simulink model "induction_motor_foc"  (R2021a)
settings: Solver=FixedStepAuto  StartTime=0.0  StopTime=3  FixedStep=0.000001  RelTol=1e-3
values from neighbouring files (symbols this model uses):
  A1 = [-1/(ts*sig) 0 lm/(ls*tr*sig) 0;0 -1/(ts*sig) 0 lm/(ls*tr*sig);lm/(lr*ts*sig) 0 -1/(tr*sig) 0; 0 lm/(lr*ts*sig) 0 -1/(tr*sig)]    [induction_motor_parameters.m]
  A2 = [0 1 0 0; -1 0 0 0;0 0 0 1;0 0 -1 0]    [induction_motor_parameters.m]
  A3 = [0 1/sig 0 lm/(ls*sig);-1/sig 0 -lm/(ls*sig) 0;0 -lm/(lr*sig) 0 -lm*lm/(ls*lr*sig); lm/(lr*sig) 0 lm*lm/(ls*lr*sig) 0]    [induction_motor_parameters.m]
  B = [1/(ls*sig) 0 0 0;0 1/(ls*sig) 0 0; -lm/(ls*lr*sig) 0 0 0;0 -lm/(ls*lr*sig) 0 0 ]    [induction_motor_parameters.m]
  fr = 0.0015    [induction_motor_parameters.m]
  j = 0.0056    [induction_motor_parameters.m]
  KiF = 2*(Rouf^2)*lr/(lm*rr)    (= 6305.05825519)    [induction_motor_parameters.m]
  KiI = 2*(Rou^2)*ls*sig    (= 315.492957746)    [induction_motor_parameters.m]
  KiV = 2*(RouV^2)*j/p    (= 0.005054)    [induction_motor_parameters.m]
  KpF = (2*Rouf-Pr)*lr/(lm*rr)    (= 111.608411481)    [induction_motor_parameters.m]
  KpI = (2*Rou-Ps)*sig*ls    (= 1.14246478873)    [induction_motor_parameters.m]
  KpV = 12*KpV    (= 0.05484)    [induction_motor_parameters.m]
  L = [ls 0 lm 0;0 ls 0 lm;lm 0 lr 0;0 lm 0 lr]    [induction_motor_parameters.m]
  lm = 0.069    [induction_motor_parameters.m]
  lr = 0.071    [induction_motor_parameters.m]
  p = 2    [induction_motor_parameters.m]
  T = [2/3 -1/3 -1/3 ; -1/3 2/3 -1/3;-1/3 -1/3 2/3]    [induction_motor_parameters.m]
  T_dent = t/m    (= 0.000952380952381)    [induction_motor_parameters.m]
  tr = lr/rr    (= 0.0870098039216)    [induction_motor_parameters.m]
libraries: simulink x4, pid_lib x4, spsdq0toabcLib x2, spsabctodq0Lib x1

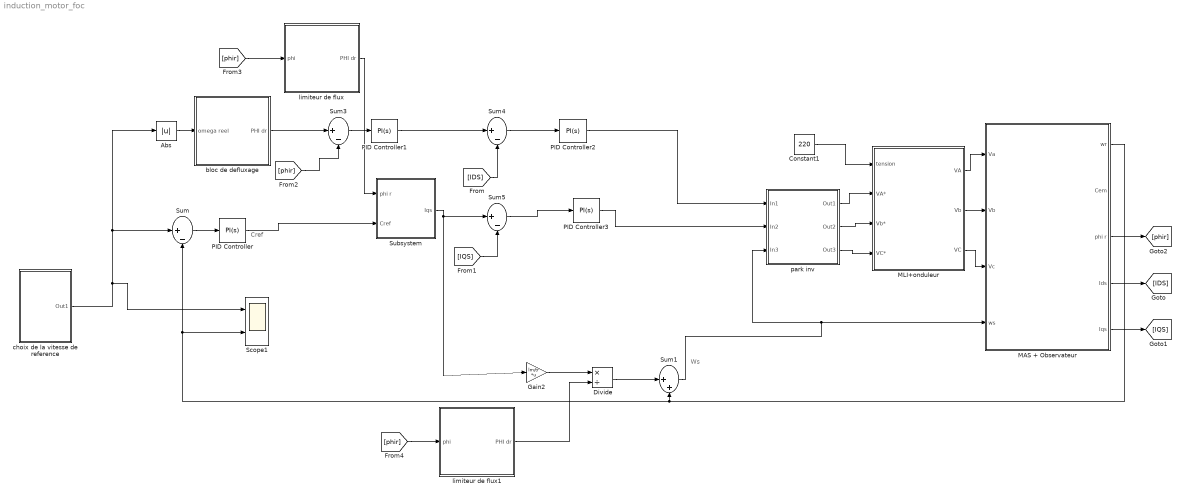
== system induction_motor_foc ==
  note: Ws
  note: Cref
  Abs : Abs
  Constant1 : Constant  Value=220
  Divide : Product  Inputs=*/
  Gain2 : Gain  Gain=lm/tr  Multiplication=Matrix(K*u)
  MAS + Observateur : Subsystem
  MLI+onduleur : Subsystem
  PID Controller : pid_lib/PID Controller  Controller=PI  Form=Parallel  TimeDomain=Continuous-time  UseExternalTs=off  SampleTime=-1  IntegratorMethod=Forward Euler  FilterMethod=Forward Euler  ControllerParametersSource=internal  P=1.7*KpV  I=KiV  D=5  UseFilter=on  N=100  TunerSelectOption=Transfer Function Based (PID Tuner App)  InitialConditionSource=internal  InitialConditionForIntegrator=0  InitialConditionForFilter=0  DifferentiatorICPrevScaledInput=0  ExternalReset=none  TrackingMode=off  Kt=1  LimitOutput=off  SatLimitsSource=internal  UpperSaturationLimit=inf  LowerSaturationLimit=-inf  LinearizeAsGain=on  AntiWindupMode=none  Kb=1  POutMin=[]  POutMax=[]  IOutMin=[]  IOutMax=[]  DOutMin=[]  DOutMax=[]  NOutMin=[]  NOutMax=[]  SumOutMin=[]  SumOutMax=[]  SaturationOutMin=[]  SaturationOutMax=[]  PParamMin=[]  PParamMax=[]  IParamMin=[]  IParamMax=[]  DParamMin=[]  DParamMax=[]  NParamMin=[]  NParamMax=[]  KbParamMin=[]  KbParamMax=[]  KtParamMin=[]  KtParamMax=[]  KbOutMin=[]  KbOutMax=[]  KtOutMin=[]  KtOutMax=[]  IntegratorOutMin=[]  IntegratorOutMax=[]  FilterOutMin=[]  FilterOutMax=[]  SumI1OutMin=[]  SumI1OutMax=[]  SumI2OutMin=[]  SumI2OutMax=[]  SumI3OutMin=[]  SumI3OutMax=[]  SumI4OutMin=[]  SumI4OutMax=[]  SumDOutMin=[]  SumDOutMax=[]  DifferentiatorOutMin=[]  DifferentiatorOutMax=[]  FilterDiffOutCoefMin=[]  FilterDiffOutCoefMax=[]  ReciprocalOutMin=[]  ReciprocalOutMax=[]  SumDenOutMin=[]  SumDenOutMax=[]  SumNumOutMin=[]  SumNumOutMax=[]  DivideOutMin=[]  DivideOutMax=[]  UdiffTsProdOutMin=[]  UdiffTsProdOutMax=[]  NTsProdOutMin=[]  NTsProdOutMax=[]  UintegralTsProdOutMin=[]  UintegralTsProdOutMax=[]  UngainTsProdOutMin=[]  UngainTsProdOutMax=[]  IntegratorContinuousStateAttributes=''  IntegratorStateMustResolveToSignalObject=off  IntegratorRTWStateStorageClass=Auto  FilterContinuousStateAttributes=''  FilterStateMustResolveToSignalObject=off  FilterRTWStateStorageClass=Auto  ParallelPVariant=InternalParameters  IdealPVariant=Disabled  IVariant=InternalParameters  DVariant=Disabled  IntegratorVariant=Continuous  SatVariant=Disabled  AWVariant=Passthrough  PCopyVariant=Disabled  TRVariant=Disabled  FdbkBlocksVariant=Forward  IdealPFdbkVariant=Disabled  SatFdbkVariant=Disabled  DerivativeFilterVariant=Disabled  NVariant=Disabled  NCopyVariant=Disabled_SignalSpec  FilterICVariant=Disabled  IntegratorICVariant=InternalICs  ExternalResetVariant=Disabled  TRSumVariant=Passthrough  SumFdbkVariant=Disabled  SumVariant=Sum_PI  TsampFilterVariant=InternalTs  TsampNgainVariant=Passthrough  TsampIntegralVariant=Passthrough  ExternalSaturationOutDataTypeStr=Inherit: Same as second input
  PID Controller1 : pid_lib/PID Controller  Controller=PI  Form=Parallel  TimeDomain=Continuous-time  UseExternalTs=off  SampleTime=-1  IntegratorMethod=Forward Euler  FilterMethod=Forward Euler  ControllerParametersSource=internal  P=KpF  I=KiF  D=0.05  UseFilter=on  N=100  TunerSelectOption=Transfer Function Based (PID Tuner App)  InitialConditionSource=internal  InitialConditionForIntegrator=0  InitialConditionForFilter=0  DifferentiatorICPrevScaledInput=0  ExternalReset=none  TrackingMode=off  Kt=1  LimitOutput=off  SatLimitsSource=internal  UpperSaturationLimit=inf  LowerSaturationLimit=-inf  LinearizeAsGain=on  AntiWindupMode=none  Kb=1  POutMin=[]  POutMax=[]  IOutMin=[]  IOutMax=[]  DOutMin=[]  DOutMax=[]  NOutMin=[]  NOutMax=[]  SumOutMin=[]  SumOutMax=[]  SaturationOutMin=[]  SaturationOutMax=[]  PParamMin=[]  PParamMax=[]  IParamMin=[]  IParamMax=[]  DParamMin=[]  DParamMax=[]  NParamMin=[]  NParamMax=[]  KbParamMin=[]  KbParamMax=[]  KtParamMin=[]  KtParamMax=[]  KbOutMin=[]  KbOutMax=[]  KtOutMin=[]  KtOutMax=[]  IntegratorOutMin=[]  IntegratorOutMax=[]  FilterOutMin=[]  FilterOutMax=[]  SumI1OutMin=[]  SumI1OutMax=[]  SumI2OutMin=[]  SumI2OutMax=[]  SumI3OutMin=[]  SumI3OutMax=[]  SumI4OutMin=[]  SumI4OutMax=[]  SumDOutMin=[]  SumDOutMax=[]  DifferentiatorOutMin=[]  DifferentiatorOutMax=[]  FilterDiffOutCoefMin=[]  FilterDiffOutCoefMax=[]  ReciprocalOutMin=[]  ReciprocalOutMax=[]  SumDenOutMin=[]  SumDenOutMax=[]  SumNumOutMin=[]  SumNumOutMax=[]  DivideOutMin=[]  DivideOutMax=[]  UdiffTsProdOutMin=[]  UdiffTsProdOutMax=[]  NTsProdOutMin=[]  NTsProdOutMax=[]  UintegralTsProdOutMin=[]  UintegralTsProdOutMax=[]  UngainTsProdOutMin=[]  UngainTsProdOutMax=[]  IntegratorContinuousStateAttributes=''  IntegratorStateMustResolveToSignalObject=off  IntegratorRTWStateStorageClass=Auto  FilterContinuousStateAttributes=''  FilterStateMustResolveToSignalObject=off  FilterRTWStateStorageClass=Auto  ParallelPVariant=InternalParameters  IdealPVariant=Disabled  IVariant=InternalParameters  DVariant=Disabled  IntegratorVariant=Continuous  SatVariant=Disabled  AWVariant=Passthrough  PCopyVariant=Disabled  TRVariant=Disabled  FdbkBlocksVariant=Forward  IdealPFdbkVariant=Disabled  SatFdbkVariant=Disabled  DerivativeFilterVariant=Disabled  NVariant=Disabled  NCopyVariant=Disabled_SignalSpec  FilterICVariant=Disabled  IntegratorICVariant=InternalICs  ExternalResetVariant=Disabled  TRSumVariant=Passthrough  SumFdbkVariant=Disabled  SumVariant=Sum_PI  TsampFilterVariant=InternalTs  TsampNgainVariant=Passthrough  TsampIntegralVariant=Passthrough  ExternalSaturationOutDataTypeStr=Inherit: Same as second input
  PID Controller2 : pid_lib/PID Controller  Controller=PI  Form=Parallel  TimeDomain=Continuous-time  UseExternalTs=off  SampleTime=-1  IntegratorMethod=Forward Euler  FilterMethod=Forward Euler  ControllerParametersSource=internal  P=KpI  I=KiI  D=0.05  UseFilter=on  N=100  TunerSelectOption=Transfer Function Based (PID Tuner App)  InitialConditionSource=internal  InitialConditionForIntegrator=0  InitialConditionForFilter=0  DifferentiatorICPrevScaledInput=0  ExternalReset=none  TrackingMode=off  Kt=1  LimitOutput=off  SatLimitsSource=internal  UpperSaturationLimit=inf  LowerSaturationLimit=-inf  LinearizeAsGain=on  AntiWindupMode=none  Kb=1  POutMin=[]  POutMax=[]  IOutMin=[]  IOutMax=[]  DOutMin=[]  DOutMax=[]  NOutMin=[]  NOutMax=[]  SumOutMin=[]  SumOutMax=[]  SaturationOutMin=[]  SaturationOutMax=[]  PParamMin=[]  PParamMax=[]  IParamMin=[]  IParamMax=[]  DParamMin=[]  DParamMax=[]  NParamMin=[]  NParamMax=[]  KbParamMin=[]  KbParamMax=[]  KtParamMin=[]  KtParamMax=[]  KbOutMin=[]  KbOutMax=[]  KtOutMin=[]  KtOutMax=[]  IntegratorOutMin=[]  IntegratorOutMax=[]  FilterOutMin=[]  FilterOutMax=[]  SumI1OutMin=[]  SumI1OutMax=[]  SumI2OutMin=[]  SumI2OutMax=[]  SumI3OutMin=[]  SumI3OutMax=[]  SumI4OutMin=[]  SumI4OutMax=[]  SumDOutMin=[]  SumDOutMax=[]  DifferentiatorOutMin=[]  DifferentiatorOutMax=[]  FilterDiffOutCoefMin=[]  FilterDiffOutCoefMax=[]  ReciprocalOutMin=[]  ReciprocalOutMax=[]  SumDenOutMin=[]  SumDenOutMax=[]  SumNumOutMin=[]  SumNumOutMax=[]  DivideOutMin=[]  DivideOutMax=[]  UdiffTsProdOutMin=[]  UdiffTsProdOutMax=[]  NTsProdOutMin=[]  NTsProdOutMax=[]  UintegralTsProdOutMin=[]  UintegralTsProdOutMax=[]  UngainTsProdOutMin=[]  UngainTsProdOutMax=[]  IntegratorContinuousStateAttributes=''  IntegratorStateMustResolveToSignalObject=off  IntegratorRTWStateStorageClass=Auto  FilterContinuousStateAttributes=''  FilterStateMustResolveToSignalObject=off  FilterRTWStateStorageClass=Auto  ParallelPVariant=InternalParameters  IdealPVariant=Disabled  IVariant=InternalParameters  DVariant=Disabled  IntegratorVariant=Continuous  SatVariant=Disabled  AWVariant=Passthrough  PCopyVariant=Disabled  TRVariant=Disabled  FdbkBlocksVariant=Forward  IdealPFdbkVariant=Disabled  SatFdbkVariant=Disabled  DerivativeFilterVariant=Disabled  NVariant=Disabled  NCopyVariant=Disabled_SignalSpec  FilterICVariant=Disabled  IntegratorICVariant=InternalICs  ExternalResetVariant=Disabled  TRSumVariant=Passthrough  SumFdbkVariant=Disabled  SumVariant=Sum_PI  TsampFilterVariant=InternalTs  TsampNgainVariant=Passthrough  TsampIntegralVariant=Passthrough  ExternalSaturationOutDataTypeStr=Inherit: Same as second input
  PID Controller3 : pid_lib/PID Controller  Controller=PI  Form=Parallel  TimeDomain=Continuous-time  UseExternalTs=off  SampleTime=-1  IntegratorMethod=Forward Euler  FilterMethod=Forward Euler  ControllerParametersSource=internal  P=KpI  I=KiI  D=0.05  UseFilter=on  N=100  TunerSelectOption=Transfer Function Based (PID Tuner App)  InitialConditionSource=internal  InitialConditionForIntegrator=0  InitialConditionForFilter=0  DifferentiatorICPrevScaledInput=0  ExternalReset=none  TrackingMode=off  Kt=1  LimitOutput=off  SatLimitsSource=internal  UpperSaturationLimit=inf  LowerSaturationLimit=-inf  LinearizeAsGain=on  AntiWindupMode=none  Kb=1  POutMin=[]  POutMax=[]  IOutMin=[]  IOutMax=[]  DOutMin=[]  DOutMax=[]  NOutMin=[]  NOutMax=[]  SumOutMin=[]  SumOutMax=[]  SaturationOutMin=[]  SaturationOutMax=[]  PParamMin=[]  PParamMax=[]  IParamMin=[]  IParamMax=[]  DParamMin=[]  DParamMax=[]  NParamMin=[]  NParamMax=[]  KbParamMin=[]  KbParamMax=[]  KtParamMin=[]  KtParamMax=[]  KbOutMin=[]  KbOutMax=[]  KtOutMin=[]  KtOutMax=[]  IntegratorOutMin=[]  IntegratorOutMax=[]  FilterOutMin=[]  FilterOutMax=[]  SumI1OutMin=[]  SumI1OutMax=[]  SumI2OutMin=[]  SumI2OutMax=[]  SumI3OutMin=[]  SumI3OutMax=[]  SumI4OutMin=[]  SumI4OutMax=[]  SumDOutMin=[]  SumDOutMax=[]  DifferentiatorOutMin=[]  DifferentiatorOutMax=[]  FilterDiffOutCoefMin=[]  FilterDiffOutCoefMax=[]  ReciprocalOutMin=[]  ReciprocalOutMax=[]  SumDenOutMin=[]  SumDenOutMax=[]  SumNumOutMin=[]  SumNumOutMax=[]  DivideOutMin=[]  DivideOutMax=[]  UdiffTsProdOutMin=[]  UdiffTsProdOutMax=[]  NTsProdOutMin=[]  NTsProdOutMax=[]  UintegralTsProdOutMin=[]  UintegralTsProdOutMax=[]  UngainTsProdOutMin=[]  UngainTsProdOutMax=[]  IntegratorContinuousStateAttributes=''  IntegratorStateMustResolveToSignalObject=off  IntegratorRTWStateStorageClass=Auto  FilterContinuousStateAttributes=''  FilterStateMustResolveToSignalObject=off  FilterRTWStateStorageClass=Auto  ParallelPVariant=InternalParameters  IdealPVariant=Disabled  IVariant=InternalParameters  DVariant=Disabled  IntegratorVariant=Continuous  SatVariant=Disabled  AWVariant=Passthrough  PCopyVariant=Disabled  TRVariant=Disabled  FdbkBlocksVariant=Forward  IdealPFdbkVariant=Disabled  SatFdbkVariant=Disabled  DerivativeFilterVariant=Disabled  NVariant=Disabled  NCopyVariant=Disabled_SignalSpec  FilterICVariant=Disabled  IntegratorICVariant=InternalICs  ExternalResetVariant=Disabled  TRSumVariant=Passthrough  SumFdbkVariant=Disabled  SumVariant=Sum_PI  TsampFilterVariant=InternalTs  TsampNgainVariant=Passthrough  TsampIntegralVariant=Passthrough  ExternalSaturationOutDataTypeStr=Inherit: Same as second input
  Scope1 : Scope  NumInputPorts=2
  Subsystem : Subsystem
  Sum{,3..5} (4 alike) : Sum  Inputs=|+-
  Sum1 : Sum  Inputs=|++
  bloc de defluxage : Subsystem
  choix de la vitesse de reference : Subsystem
  limiteur de flux : Subsystem
  limiteur de flux1 : Subsystem
  park inv : Subsystem
  wires:
  MLI+onduleur/1(VA) -> MAS + Observateur/1(Va)
  Sum/1 -> PID Controller/1
  [IDS] -> Sum4/2
  MAS + Observateur/5(Iqs) -> [IQS]
  Sum4/1 -> PID Controller2/1
  Divide/1 -> Sum1/1
  MLI+onduleur/3(VC) -> MAS + Observateur/3(Vc)
  Sum1/1 -> park inv/3(In3), MAS + Observateur/4(ws)
  Sum5/1 -> PID Controller3/1
  MAS + Observateur/4(Ids) -> [IDS]
  MLI+onduleur/2(Vb) -> MAS + Observateur/2(Vb)
  PID Controller3/1 -> park inv/2(In2)
  park inv/3(Out3) -> MLI+onduleur/4(VC*)
  PID Controller2/1 -> park inv/1(In1)
  Constant1/1 -> MLI+onduleur/1(tension)
  Subsystem/1(Iqs) -> Sum5/1, Gain2/1
  park inv/1(Out1) -> MLI+onduleur/2(VA*)
  bloc de defluxage/1(PHI dr) -> Sum3/1
  park inv/2(Out2) -> MLI+onduleur/3(Vb*)
  Gain2/1 -> Divide/1
  PID Controller/1 -> Subsystem/2(Cref)
  MAS + Observateur/1(wr) -> Sum1/2, Sum/2, Scope1/2
  [IQS] -> Sum5/2
  PID Controller1/1 -> Sum4/1
  Sum3/1 -> PID Controller1/1
  MAS + Observateur/3(phi r) -> [phir]
  [phir] -> Sum3/2
  [phir] -> limiteur de flux/1(phi)
  limiteur de flux/1(PHI dr) -> Subsystem/1(phi r)
  Abs/1 -> bloc de defluxage/1(omega reel)
  limiteur de flux1/1(PHI dr) -> Divide/2
  [phir] -> limiteur de flux1/1(phi)
  choix de la vitesse de reference/1(Out1) -> Abs/1, Sum/1, Scope1/1

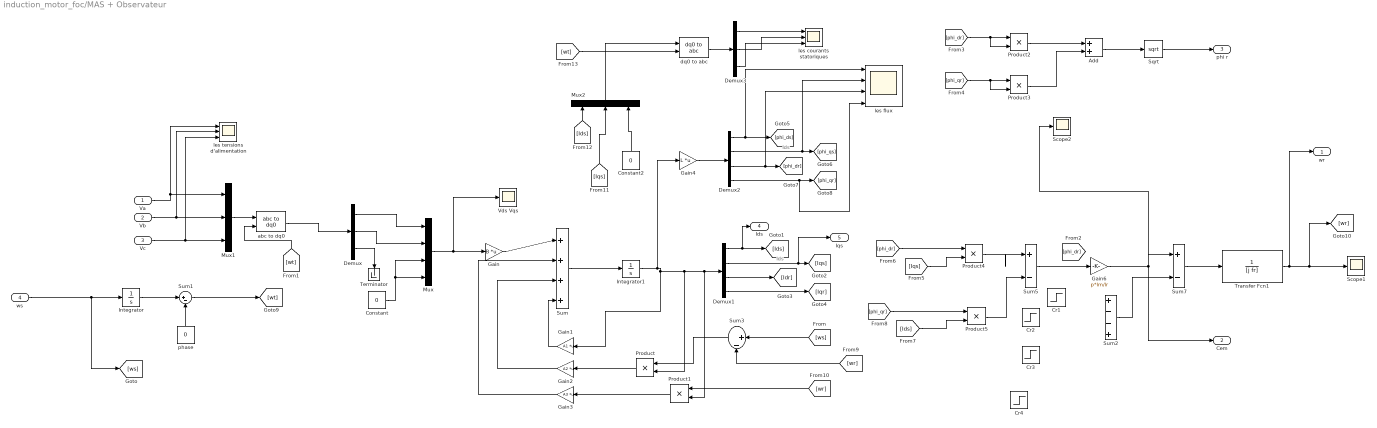
== system induction_motor_foc/MAS + Observateur ==
  note: Ids
  note: Ids
  Va : Inport
  Vb : Inport  Port=2
  Vc : Inport  Port=3
  ws : Inport  Port=4
  Add : Sum
  Constant : Constant  Value=0
  Constant2 : Constant  Value=0
  Cr1 : Step  After=5  SampleTime=0
  Cr2 : Step  Time=1.01  After=5  SampleTime=0
  Cr3 : Step  Time=1.5  After=5  SampleTime=0
  Cr4 : Step  Time=1.51  After=5  SampleTime=0
  Demux : Demux  Outputs=3
  Demux1 : Demux
  Demux2 : Demux
  Demux3 : Demux  Outputs=3
  Gain : Gain  Gain=B  Multiplication=Matrix(K*u)
  Gain1 : Gain  Gain=A1  Multiplication=Matrix(K*u)
  Gain2 : Gain  Gain=A2  Multiplication=Matrix(K*u)
  Gain3 : Gain  Gain=A3  Multiplication=Matrix(K*u)
  Gain4 : Gain  Gain=L  Multiplication=Matrix(K*u)
  Gain6 : Gain  Gain=p*lm/lr
  Integrator : Integrator
  Integrator1 : Integrator
  Mux : Mux
  Mux1 : Mux  Inputs=3
  Mux2 : Mux  Inputs=3
  Product{,1..5} (6 alike) : Product
  Scope1 : Scope
  Scope2 : Scope
  Sqrt : Sqrt  SaturateOnIntegerOverflow=on
  Sum : Sum  Inputs=|++++
  Sum{1,3,5,7} (4 alike) : Sum  Inputs=|+-
  Sum2 : Sum  Inputs=|+--+
  Terminator : Terminator
  Transfer Fcn1 : TransferFcn  Denominator=[j fr]
  Vds Vqs : Scope
  abc to dq0 : spsabctodq0Lib/abc to dq0  Alignment=Aligned with phase A axis
  dq0 to abc : spsdq0toabcLib/dq0 to abc  Alignment=90 degrees behind phase A axis
  les courants statoriques : Scope  NumInputPorts=3
  les flux : Scope  NumInputPorts=4
  "les tensions d'alimentation " : Scope  NumInputPorts=3
  phase : Constant  Value=0
  wr : Outport
  Cem : Outport  Port=2
  phi r : Outport  Port=3
  Ids : Outport  Port=4
  Iqs : Outport  Port=5
  wires:
  Product/1 -> Gain2/1
  [wr] -> Product1/1
  Transfer Fcn1/1 -> wr/1, [wr], Scope1/1
  Demux2/1 -> les flux/1, [phi_ds]
  Gain2/1 -> Sum/3
  Gain/1 -> Sum/1
  Constant2/1 -> Mux2/3
  Sum3/1 -> Product/1
  [Iqs] -> Product4/2
  Gain4/1 -> Demux2/1
  Demux2/3 -> les flux/3, [phi_dr]
  [wt] -> dq0 to abc/2
  Constant/1 -> Mux/4, Mux/3
  [phi_dr] -> Product4/1
  phase/1 -> Sum1/2
  Integrator1/1 -> Gain4/1, Product/2, Product1/2, Demux1/1, Gain1/1
  Demux/3 -> Terminator/1
  Demux/2 -> Mux/2
  [ws] -> Sum3/1
  Demux2/2 -> les flux/2, [phi_qs]
  Integrator/1 -> Sum1/1
  Demux1/4 -> [Iqr]
  Demux1/3 -> [Idr]
  Demux1/1 -> Ids/1, [Ids]
  Sum1/1 -> [wt]
  Gain3/1 -> Sum/2
  Mux/1 -> Vds Vqs/1, Gain/1
  Gain6/1 -> Cem/1, Scope2/1, Sum7/1
  Product1/1 -> Gain3/1
  Mux2/1 -> dq0 to abc/1
  Gain1/1 -> Sum/4
  [wr] -> Sum3/2
  Sum7/1 -> Transfer Fcn1/1
  Sum5/1 -> Gain6/1
  [Ids] -> Product5/2
  [phi_qr] -> Product5/1
  Demux1/2 -> Iqs/1, [Iqs]
  Demux/1 -> Mux/1
  Sum/1 -> Integrator1/1
  Product4/1 -> Sum5/1
  Product5/1 -> Sum5/2
  [Iqs] -> Mux2/2
  [Ids] -> Mux2/1
  ws/1 -> Integrator/1, [ws]
  Va/1 -> "les tensions d'alimentation "/1, Mux1/1
  Vc/1 -> "les tensions d'alimentation "/3, Mux1/3
  Mux1/1 -> abc to dq0/1
  [wt] -> abc to dq0/2
  abc to dq0/1 -> Demux/1
  [phi_dr] -> Product2/2, Product2/1
  [phi_qr] -> Product3/2, Product3/1
  Product2/1 -> Add/1
  Product3/1 -> Add/2
  Add/1 -> Sqrt/1
  Sqrt/1 -> phi r/1
  Demux2/4 -> les flux/4, [phi_qr]
  dq0 to abc/1 -> Demux3/1
  Demux3/1 -> les courants statoriques/1
  Demux3/2 -> les courants statoriques/2
  Demux3/3 -> les courants statoriques/3
  Sum2/1 -> Sum7/2
  Vb/1 -> "les tensions d'alimentation "/2, Mux1/2

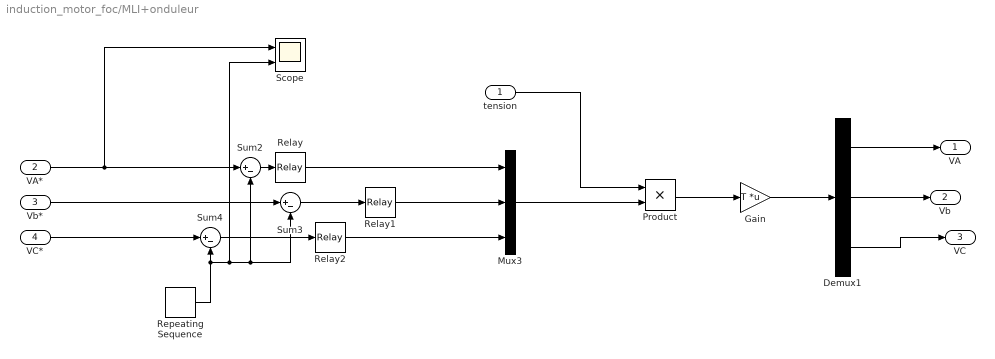
== system induction_motor_foc/MLI+onduleur ==
  tension : Inport
  VA* : Inport  Port=2
  Vb* : Inport  Port=3
  VC* : Inport  Port=4
  Demux1 : Demux  Outputs=3
  Gain : Gain  Gain=T  Multiplication=Matrix(K*u)
  Mux3 : Mux  Inputs=3
  Product : Product
  Relay : Relay  OffOutputValue=-1
  Relay1 : Relay  OffOutputValue=-1
  Relay2 : Relay  OffOutputValue=-1
  Repeating Sequence : simulink/Sources/Repeating Sequence  rep_seq_t="[0  T_dent/2 T_dent ]"  rep_seq_y=[-350 350 -350]
  Scope : Scope  NumInputPorts=2
  Sum2 : Sum  Inputs=|+-
  Sum3 : Sum  Inputs=|+-
  Sum4 : Sum  Inputs=|+-
  VA : Outport
  Vb : Outport  Port=2
  VC : Outport  Port=3
  wires:
  Relay/1 -> Mux3/1
  Repeating Sequence/1 -> Scope/2, Sum2/2, Sum3/2, Sum4/2
  Product/1 -> Gain/1
  Relay1/1 -> Mux3/2
  Sum3/1 -> Relay1/1
  Mux3/1 -> Product/2
  Relay2/1 -> Mux3/3
  Sum2/1 -> Relay/1
  Sum4/1 -> Relay2/1
  Gain/1 -> Demux1/1
  tension/1 -> Product/1
  Vb*/1 -> Sum3/1
  Demux1/2 -> Vb/1
  VC*/1 -> Sum4/1
  VA*/1 -> Scope/1, Sum2/1
  Demux1/3 -> VC/1
  Demux1/1 -> VA/1

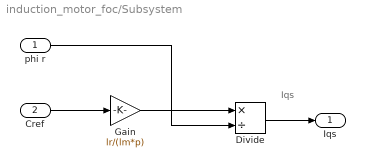
== system induction_motor_foc/Subsystem ==
  note: Iqs
  phi r : Inport
  Cref : Inport  Port=2
  Divide : Product  Inputs=*/
  Gain : Gain  Gain=lr/(lm*p)
  Iqs : Outport
  wires:
  phi r/1 -> Divide/2
  Divide/1 -> Iqs/1
  Cref/1 -> Gain/1
  Gain/1 -> Divide/1

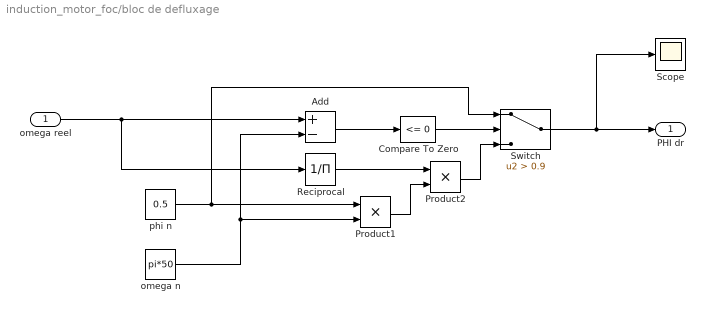
== system induction_motor_foc/bloc de defluxage ==
  omega reel : Inport
  Add : Sum  Inputs=+-
  Compare To Zero : simulink/Logic and Bit Operations/Compare To Zero  relop=<=  OutDataTypeStr=boolean
  Product1 : Product
  Product2 : Product
  Reciprocal : Product  Inputs=/
  Scope : Scope
  Switch : Switch  Criteria=u2 > Threshold  Threshold=0.9
  omega n : Constant  Value=pi*50
  phi n : Constant  Value=0.5
  PHI dr : Outport
  wires:
  omega reel/1 -> Reciprocal/1, Add/1
  omega n/1 -> Product1/2, Add/2
  Product2/1 -> Switch/3
  phi n/1 -> Switch/1, Product1/1
  Add/1 -> Compare To Zero/1
  Reciprocal/1 -> Product2/1
  Compare To Zero/1 -> Switch/2
  Product1/1 -> Product2/2
  Switch/1 -> Scope/1, PHI dr/1

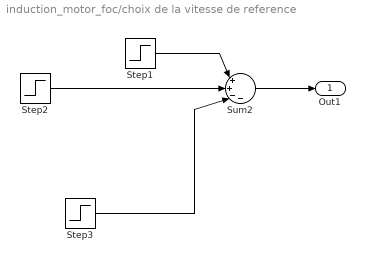
== system induction_motor_foc/choix de la vitesse de reference ==
  Step1 : Step  Time=0.5  After=100  SampleTime=0
  Step2 : Step  Time=1.5  After=50  SampleTime=0
  Step3 : Step  Time=2  After=250  SampleTime=0
  Sum2 : Sum  Inputs=|++--
  Out1 : Outport
  wires:
  Step1/1 -> Sum2/1
  Sum2/1 -> Out1/1
  Step3/1 -> Sum2/3
  Step2/1 -> Sum2/2

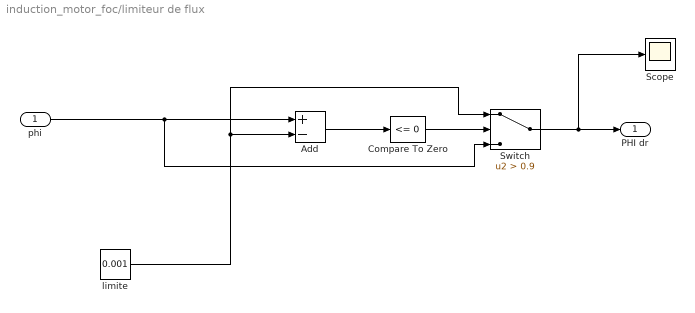
== system induction_motor_foc/limiteur de flux ==
  phi : Inport
  Add : Sum  Inputs=+-
  Compare To Zero : simulink/Logic and Bit Operations/Compare To Zero  relop=<=  OutDataTypeStr=boolean
  Scope : Scope
  Switch : Switch  Criteria=u2 > Threshold  Threshold=0.9
  limite : Constant  Value=0.001
  PHI dr : Outport
  wires:
  phi/1 -> Switch/3, Add/1
  limite/1 -> Switch/1, Add/2
  Add/1 -> Compare To Zero/1
  Compare To Zero/1 -> Switch/2
  Switch/1 -> Scope/1, PHI dr/1

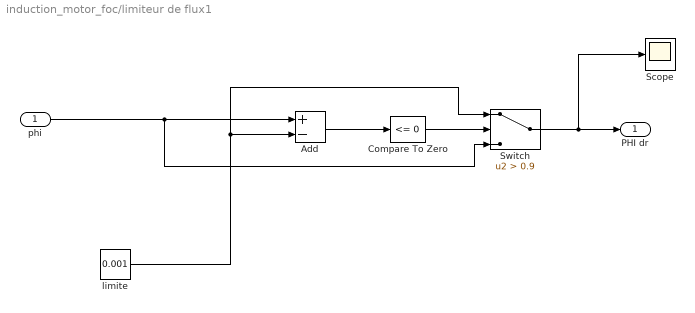
== system induction_motor_foc/limiteur de flux1 ==
  phi : Inport
  Add : Sum  Inputs=+-
  Compare To Zero : simulink/Logic and Bit Operations/Compare To Zero  relop=<=  OutDataTypeStr=boolean
  Scope : Scope
  Switch : Switch  Criteria=u2 > Threshold  Threshold=0.9
  limite : Constant  Value=0.001
  PHI dr : Outport
  wires:
  phi/1 -> Switch/3, Add/1
  limite/1 -> Switch/1, Add/2
  Add/1 -> Compare To Zero/1
  Compare To Zero/1 -> Switch/2
  Switch/1 -> Scope/1, PHI dr/1

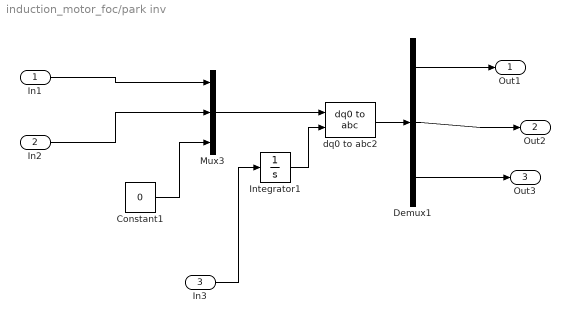
== system induction_motor_foc/park inv ==
  In1 : Inport
  In2 : Inport  Port=2
  In3 : Inport  Port=3
  Constant1 : Constant  Value=0
  Demux1 : Demux  Outputs=3
  Integrator1 : Integrator
  Mux3 : Mux  Inputs=3
  dq0 to abc2 : spsdq0toabcLib/dq0 to abc  Alignment=Aligned with phase A axis
  Out1 : Outport
  Out2 : Outport  Port=2
  Out3 : Outport  Port=3
  wires:
  dq0 to abc2/1 -> Demux1/1
  In1/1 -> Mux3/1
  Mux3/1 -> dq0 to abc2/1
  Constant1/1 -> Mux3/3
  Demux1/3 -> Out3/1
  Integrator1/1 -> dq0 to abc2/2
  In3/1 -> Integrator1/1
  Demux1/1 -> Out1/1
  In2/1 -> Mux3/2
  Demux1/2 -> Out2/1
